simulink model "gm_comm8qamtxrxhdl"  (R2025b)
settings: Solver=FixedStepDiscrete  StartTime=0.0  StopTime=20000*qam_params.symbolPeriod  RelTol=1e-3
PreLoadFcn:
  | qam_params = comm8qamtxrxhdl_init;
InitFcn:
  | qam_params = comm8qamtxrxhdl_init;
libraries: simulink x16, hdlmdlgenlib x7, hdlsllib x7, commchan3 x1, commrflib2 x1, dspsigops x1, dsphdlsigops2 x1, dspmlti4 x1, commdigbbndam3 x1, commsequence2 x1
(part 1 of 3)
settings Model: Creator=The MathWorks, Inc.  LastModifiedBy=Ubaid
settings SolverCC: AlgebraicLoopSolver=TrustRegion  MaxZcPerStep=1.0
settings DataIOCC: LimitDataPoints=on  SaveFormat=Array  SaveOutput=off  SaveTime=off  ReturnWorkspaceOutputs=off
settings OptimizationCC: BlockReduction=off  ConditionallyExecuteInputs=off  DefaultParameterBehavior=Inlined  ReuseModelBlockBuffer=off  LifeSpan=inf
settings DebuggingCC: AlgebraicLoopMsg=error  ArtificialAlgebraicLoopMsg=none  UnderspecifiedInitializationDetection=Classic  MergeDetectMultiDrivingBlocksExec=none  SolverPrmCheckMsg=warning  InheritedTsInSrcMsg=none  MultiTaskDSMMsg=warning  MultiTaskCondExecSysMsg=none  SingleTaskRateTransMsg=error  IntegerOverflowMsg=none  ParameterPrecisionLossMsg=none  UnconnectedInputMsg=warning  UnconnectedOutputMsg=warning  UnconnectedLineMsg=warning  AllowSymbolicDim=off  StateNameClashWarn=warning  SFUnexpectedBacktrackingDiag=warning  SFNoUnconditionalDefaultTransitionDiag=warning  SFExecutionAtInitializationDiag=none  IntegerSaturationMsg=none  ArithmeticOperatorsInVariantConditions=warning
settings HardwareCC: ProdBitPerPointer=32.0  ProdBitPerSizeT=32.0  ProdBitPerPtrDiffT=32.0  ProdLargestAtomicFloat=None  ProdIntDivRoundTo=Undefined  ProdEndianess=Unspecified  ProdWordSize=32.0  ProdHWDeviceType=ASIC/FPGA->ASIC/FPGA  ProdEqTarget=off
settings ModelReferenceCC: EnableRefExpFcnMdlSchedulingChecks=on  PropagateSignalLabelsOutOfModel=off
settings SFSimCC: SimUseLocalCustomCode=off  CustomCodeUndefinedFunction=UseInterfaceOnly
settings RTWCC: RTWUseLocalCustomCode=off  GPUComputeCapability=3.5  DLArmComputeVersion=19.05
settings CodeAppCC: StateflowObjectComments=on
settings GRTTargetCC: TargetLangStandard=C89/C90 (ANSI)
settings ConfigComp: CovMetricSettings=dw  CovSaveCumulativeToWorkspaceVar=on  CovSaveSingleToWorkspaceVar=on  CovExternalEMLEnable=off  CovSFcnEnable=off

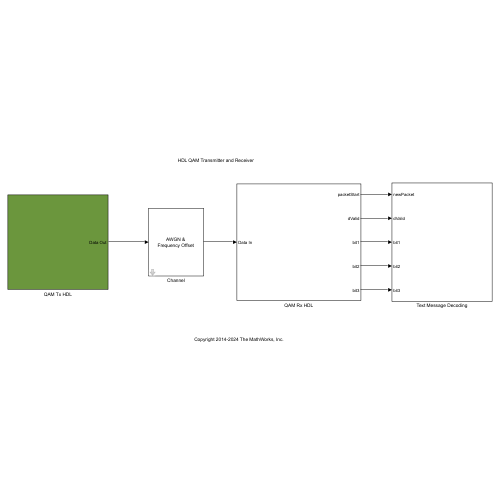
[thumbnail: Simulink's stored preview of the top-level diagram]
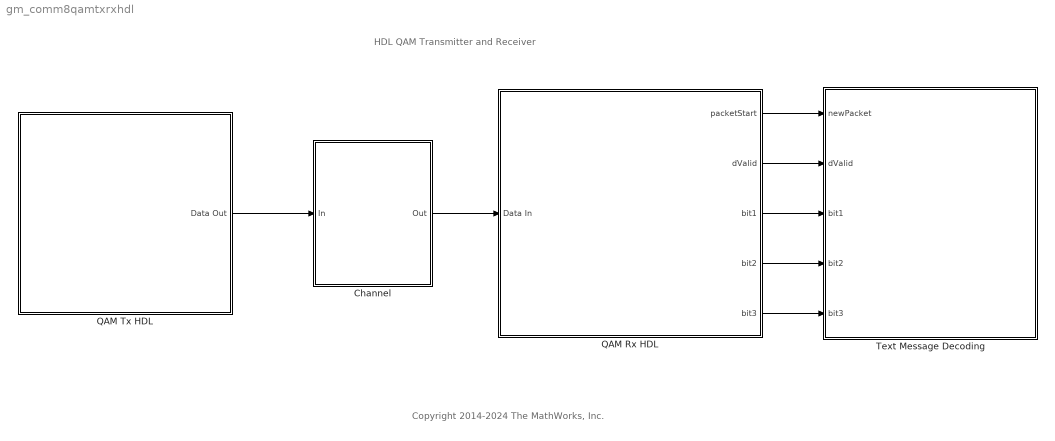
== system gm_comm8qamtxrxhdl ==
  note: HDL QAM Transmitter and Receiver
  note: Copyright 2014-2024 The MathWorks, Inc.
  Channel : Subsystem  mask{Poff=qam_params.phaseOffset, Foff=qam_params.frequencyOffset, EbNo=qam_params.EbNo, Chan_Gain=qam_params.channelGain, Chan_Delay=qam_params.channelDelay}
      mask prompts: Poff "Phase offset (deg)"; Foff "Frequency offset (Hz)"; EbNo "Eb/No"; Chan_Gain "Channel Gain"; Chan_Delay "Channel Delay"
      mask Display: disp('AWGN &\nFrequency Offset');
  QAM Rx HDL : Subsystem
  QAM Tx HDL : Subsystem
  Text Message Decoding : Subsystem
  wires:
  QAM Tx HDL/1(Data Out) -> Channel/1(In)
  Channel/1(Out) -> QAM Rx HDL/1(Data In)
  QAM Rx HDL/2(dValid) -> Text Message Decoding/2(dValid)
  QAM Rx HDL/5(bit3) -> Text Message Decoding/5(bit3)
  QAM Rx HDL/4(bit2) -> Text Message Decoding/4(bit2)
  QAM Rx HDL/3(bit1) -> Text Message Decoding/3(bit1)
  QAM Rx HDL/1(packetStart) -> Text Message Decoding/1(newPacket)

== system gm_comm8qamtxrxhdl/Channel ==
  In : Inport
  AWGN Channel2 : commchan3/AWGN Channel  LegacyMode=on  NoiseMethod="Signal to noise ratio  (Eb/No)"  noiseMode="Signal to noise ratio  (SNR)"  EbNo=EbNo  EsNo=15  SNR=15  BitsPerSymbol=3  SignalPower=0.11  SpecifySymbolPeriod=off  SamplesPerSymbol=1  SymbolPeriod=1/qam_params.sampleRate  VarianceSource=Parameter  Variance=1  RandomStream=Global stream  Seed=67  SimulateUsing=Code generation
  Constant : Constant  Value=Chan_Delay  SampleTime=1/qam_params.sampleRate
  Data Type Conversion1 : DataTypeConversion  OutDataTypeStr=fixdt(1,16,15)  SaturateOnIntegerOverflow=off  RndMeth=Floor
  Data Type Conversion4 : DataTypeConversion  OutDataTypeStr=double  SaturateOnIntegerOverflow=off  RndMeth=Floor
  Gain : Gain  Gain=Chan_Gain
  Phase/ Frequency Offset1 : commrflib2/Phase// Frequency Offset  phaseOffset=Poff  freqPort=off  freqOffset=Foff
  Variable Fractional Delay : dspsigops/Variable Fractional Delay  mode=OBSOLETE  modeActive=Linear  L=4  FarrowL=4  R=10  alpha=1  dmax=56*4  ic=0  noDFT=off  fallbackFIR=Clip to the minimum value necessary for centered kernel  fallbackFarrow=Clip to the minimum value necessary for centered kernel  roundingMode=Zero  overflowMode=off
  Out : Outport  VectorParamsAs1DForOutWhenUnconnected=off
  wires:
  Gain/1 -> Data Type Conversion1/1
  Constant/1 -> Variable Fractional Delay/2
  Variable Fractional Delay/1 -> AWGN Channel2/1
  Phase/ Frequency Offset1/1 -> Variable Fractional Delay/1
  Data Type Conversion4/1 -> Phase/ Frequency Offset1/1
  Data Type Conversion1/1 -> Out/1
  AWGN Channel2/1 -> Gain/1
  In/1 -> Data Type Conversion4/1

== system gm_comm8qamtxrxhdl/QAM Rx HDL ==
  Data In : Inport  OutDataTypeStr=fixdt(1, 16, 15)  PortDimensions=1  SampleTime=2.5e-07
      settings: SignalType=complex
  AND : Logic  AllPortsSameDT=off  OutDataTypeStr=boolean  SampleTime=5e-07
  Automatic Gain Control : Subsystem  mask{AGC_Ref=double(0.23), AGC_Gain=double(0.001)}
      mask prompts: AGC_Ref "Target Amplitude"; AGC_Gain "AGC Loop Gain"
  Coarse Frequency Offset Correction : Subsystem
  Delay3 : Delay  DelayLength=double(2)  InitialCondition=0  SampleTime=5e-07
  Demodulate : Subsystem
  Magnitude & Phase Recovery : Subsystem  mask{PreAmb=reshape(complex(double([0.75+0.25i;0.75+0.25i;0.75+0.25i;0.75+0.25i;0.75+0.25i;-0.75-0.25i;-0.75-0.25i;0.75+0.25i;0.75+0.25i;-0.75-0.25i;0.75+0.25i;-0.75-0.25i;0.75+0.25i;0.75+0.25i])), [1  14]), threshold=double(1.1), LMS_Step=double(0.25)}
      mask prompts: PreAmb "Preamble symbols"; LMS_Step "LMS step size"
  Timing Recovery : Subsystem
  packetStart : Outport  SampleTime=5e-07  VectorParamsAs1DForOutWhenUnconnected=off
  dValid : Outport  Port=2  SampleTime=5e-07  VectorParamsAs1DForOutWhenUnconnected=off
  bit1 : Outport  Port=3  SampleTime=5e-07  VectorParamsAs1DForOutWhenUnconnected=off
  bit2 : Outport  Port=4  SampleTime=5e-07  VectorParamsAs1DForOutWhenUnconnected=off
  bit3 : Outport  Port=5  SampleTime=5e-07  VectorParamsAs1DForOutWhenUnconnected=off
  wires:
  Data In/1 -> Automatic Gain Control/1(x)
  Magnitude & Phase Recovery/1(valid) -> AND/2
  Timing Recovery/2(dataOut) -> Magnitude & Phase Recovery/1(Input)
  Automatic Gain Control/1(y) -> Coarse Frequency Offset Correction/1(dataIn)
  Demodulate/1(Valid) -> dValid/1
  Coarse Frequency Offset Correction/1(dataOut) -> Timing Recovery/1(dataIn)
  Magnitude & Phase Recovery/2(corrected) -> Demodulate/2(Symbols In)
  AND/1 -> Demodulate/1(valid_in)
  Timing Recovery/1(validOut) -> AND/1, Magnitude & Phase Recovery/2(Enable)
  Demodulate/3(Bit2) -> bit2/1
  Magnitude & Phase Recovery/3(isPreamble) -> Delay3/1
  Delay3/1 -> packetStart/1
  Demodulate/2(Bit1) -> bit1/1
  Demodulate/4(Bit3) -> bit3/1

== system gm_comm8qamtxrxhdl/QAM Tx HDL ==
  " Zero" : Constant  Value=complex(0,0)  OutDataTypeStr=fixdt(1,16,15)  SampleTime=qam_params.symbolPeriod
  Data Generation & Packetization : Subsystem
  Input Mux : MultiPortSwitch  DataPortOrder=Zero-based contiguous  Inputs=2  zeroidx=on  SaturateOnIntegerOverflow=off  InputSameDT=off
  Pipeline{1..5} (5 alike) : Delay  DelayLength=1  InitialCondition=0
  Pulse Shaping : Subsystem
  Symbol Mapping : Subsystem
  Data Out : Outport  VectorParamsAs1DForOutWhenUnconnected=off
  wires:
  Pulse Shaping/1(dataOut) -> Pipeline5/1
  Input Mux/1 -> Pulse Shaping/1(dataIn)
  Symbol Mapping/1(Valid out) -> Pipeline3/1
  Symbol Mapping/2(Symbol Out) -> Pipeline4/1
  Pipeline2/1 -> Symbol Mapping/2(Integer In)
  Data Generation & Packetization/2(Raw Data) -> Pipeline2/1
  Data Generation & Packetization/1(Valid Out) -> Pipeline1/1
  " Zero"/1 -> Input Mux/2
  Pipeline3/1 -> Input Mux/1
  Pipeline1/1 -> Symbol Mapping/1(Valid In)
  Pipeline5/1 -> Data Out/1
  Pipeline4/1 -> Input Mux/3

== system gm_comm8qamtxrxhdl/Text Message Decoding ==
  newPacket : Inport
  dValid : Inport  Port=2
  bit1 : Inport  Port=3
  bit2 : Inport  Port=4
  bit3 : Inport  Port=5
  " " : MATLAB Function  TreatAsAtomicUnit=on
  Descramble and Print : Subsystem  TreatAsAtomicUnit=on
  wires:
  newPacket/1 -> " "/1(newPacket)
  dValid/1 -> " "/2(dValid)
  bit3/1 -> " "/5(bit3)
  " "/1(RxGo) -> Descramble and Print/Enable
  " "/2(framed_data) -> Descramble and Print/1(In1)
  bit2/1 -> " "/4(bit2)
  bit1/1 -> " "/3(bit1)

== system gm_comm8qamtxrxhdl/QAM Rx HDL/Automatic Gain Control ==
  x : Inport  OutDataTypeStr=fixdt(1, 16, 15)  PortDimensions=1  SampleTime=2.5e-07
      settings: SignalType=complex
  Delay : Delay  DelayLength=double(2)  InitialCondition=0  SampleTime=2.5e-07
  Delay1 : Delay  DelayLength=double(2)  InitialCondition=0  SampleTime=2.5e-07
  Delay2 : Delay  DelayLength=double(1)  InitialCondition=0  SampleTime=2.5e-07
  Delay4 : Delay  DelayLength=double(2)  InitialCondition=0  SampleTime=2.5e-07
  Loop gain : Constant  Value=0.001007080078125  OutDataTypeStr=fixdt(1, 16, 15)  SampleTime=2.5e-07
  Product : Product  Inputs=**  OutDataTypeStr=fixdt(1, 16, 15)  SaturateOnIntegerOverflow=on  SampleTime=2.5e-07
  Product1 : Product  Inputs=**  OutDataTypeStr=fixdt(1, 16, 15)  SaturateOnIntegerOverflow=on  SampleTime=2.5e-07
  Reference : Constant  Value=0.230010986328125  OutDataTypeStr=fixdt(1, 16, 15)  SampleTime=2.5e-07
  Sum : Sum  OutDataTypeStr=fixdt(1, 24, 15)  AccumDataTypeStr=fixdt(1, 24, 15)  SaturateOnIntegerOverflow=on  SampleTime=2.5e-07
  Sum1 : Sum  Inputs=+-  OutDataTypeStr=fixdt(1, 16, 14)  AccumDataTypeStr=fixdt(1, 18, 15)  SampleTime=2.5e-07
  Unit Delay : Delay  DelayLength=double(1)  InitialCondition=0.5  SampleTime=2.5e-07
  power : Subsystem
  y : Outport  PortDimensions=1  SampleTime=2.5e-07  VectorParamsAs1DForOutWhenUnconnected=off
  wires:
  Delay2/1 -> Product1/1
  Reference/1 -> Sum1/1
  power/1(Out1) -> Sum1/2
  x/1 -> Delay1/1
  Sum1/1 -> Delay2/1
  Product1/1 -> Delay4/1
  Loop gain/1 -> Product1/2
  Delay4/1 -> Sum/2
  Unit Delay/1 -> Product/2, Sum/1
  Delay1/1 -> Product/1
  Sum/1 -> Unit Delay/1
  Product/1 -> Delay/1
  Delay/1 -> power/1(In1), y/1

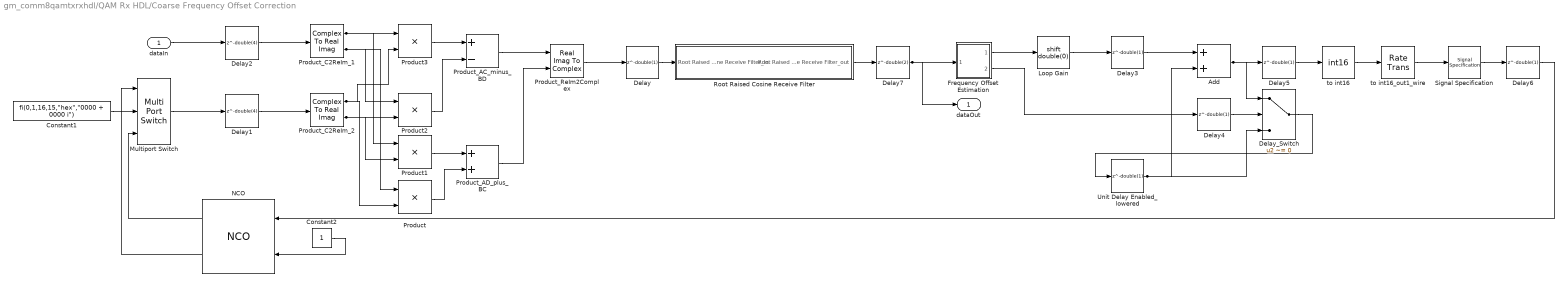
== system gm_comm8qamtxrxhdl/QAM Rx HDL/Coarse Frequency Offset Correction ==
  dataIn : Inport  OutDataTypeStr=fixdt(1, 16, 15)  PortDimensions=1  SampleTime=2.5e-07
      settings: SignalType=complex
  Add : Sum  OutDataTypeStr=fixdt(1, 16, 3)  AccumDataTypeStr=fixdt(1, 16, 3)  SampleTime=5e-07
  Constant1 : Constant  Value="fi(0,1,16,15,\"hex\",\"0000 + 0000 i\")"  OutDataTypeStr=fixdt(1, 16, 15)  SampleTime=2.5e-07
  Constant2 : Constant  OutDataTypeStr=boolean  SampleTime=2.5e-07
  Delay : Delay  DelayLength=double(1)  InitialCondition=0  SampleTime=2.5e-07
  Delay1 : Delay  DelayLength=double(4)  InitialCondition=0  SampleTime=2.5e-07
  Delay2 : Delay  DelayLength=double(4)  InitialCondition=0  SampleTime=2.5e-07
  Delay3 : Delay  DelayLength=double(1)  InitialCondition=0  SampleTime=5e-07
  Delay4 : Delay  DelayLength=double(1)  InitialCondition=0  SampleTime=5e-07
  Delay5 : Delay  DelayLength=double(1)  InitialCondition=0  SampleTime=5e-07
  Delay6 : Delay  DelayLength=double(1)  InitialCondition=0  SampleTime=2.5e-07
  Delay7 : Delay  DelayLength=double(2)  InitialCondition=0  SampleTime=5e-07
  Delay_Switch : Switch  Criteria=u2 ~= 0  Threshold=double(0)  OutDataTypeStr=fixdt(1, 16, 3)  SampleTime=5e-07  SaturateOnIntegerOverflow=off  InputSameDT=off
  Frequency Offset Estimation : Subsystem  mask{M=double(64), N=double(256), avFilterCoeffs=double(0)}
      mask prompts: M "M (Luise Parameter)"; N "N (Luise Parameter)"; avFilterCoeffs "Filter Coeffs"
      mask init:
      | M = double(64);
      | N = double(256);
      | avFilterCoeffs = reshape(double([0.00390625;0.00390625;0.00390625;0.00390625;0.00390625;0.00390625;0.00390625;0.00390625;0.00390625;0.00390625;0.00390625;0.00390625;0.00390625;0.00390625;0.00390625;0.00390625;0.00390625;0.00390625;0.00390625;0.00390625;0.00390625;0.00390625;0.00390625;0.00390625;0.00390625;0.00390625;0.00390625;0.00390625;0.00390625;0.00390625;0.00390625;0.00390625;0.00390625;0.00390625;0.00390625;0.00390625;0.00390625;0.00390625;0.00390625;0.00390625;0.00390625;0.00390625;0.00390625;0.00390625;0.00390625;0.00390625;0.00390625;0.00390625;0.00390625;0.00390625;0.00390625;0.00390625;0.00390625;0.00390625;0.00390625;0.00390625;0.00390625;0.00390625;0.00390625;0.00390625;0.00390625;0.00390625;0.00390625;0.00390625]), [1  64]);
  Loop Gain : ArithShift  BitShiftNumber=double(0)  BinPtShiftNumber=double(-3)
  Multiport Switch : MultiPortSwitch  DataPortOrder=Zero-based contiguous  Inputs=2  DiagnosticForDefault=None  zeroidx=on  OutDataTypeStr=fixdt(1, 16, 15)  SampleTime=2.5e-07  SaturateOnIntegerOverflow=off  InputSameDT=off
  NCO : dsphdlsigops2/NCO  PhaseIncrementSource=Input port  PhaseIncrement=100  PhaseOffsetSource=Property  PhaseOffset=0  DitherSource=Property  NumDitherBits=4  SamplesPerFrame=1  LUTCompress=off  ResetAction=off  Waveform=Complex exponential  PhasePort=off  SimulateUsing=Code generation  AccumulatorWL=16  PhaseQuantization=on  NumQuantizerAccumulatorBits=16  OutputDataType=Binary point scaling  OutputWL=16  OutputFL=15
  Product{,1..3} (4 alike) : Product  Inputs=**  OutDataTypeStr=fixdt(1, 16, 15)  SampleTime=2.5e-07
  Product_AC_minus_BD : Sum  Inputs=+-  OutDataTypeStr=fixdt(1, 16, 15)  SampleTime=2.5e-07
  Product_AD_plus_BC : Sum  OutDataTypeStr=fixdt(1, 16, 15)  SampleTime=2.5e-07
  Product_C2ReIm_1 : ComplexToRealImag  SampleTime=2.5e-07
  Product_C2ReIm_2 : ComplexToRealImag  SampleTime=2.5e-07
  Product_ReIm2Complex : RealImagToComplex  SampleTime=2.5e-07
  Root Raised Cosine Receive Filter : Subsystem
  Signal Specification : SignalSpecification  OutDataTypeStr=int16  Dimensions=1
  Unit Delay Enabled_lowered : Delay  DelayLength=double(1)  InitialCondition=0  SampleTime=5e-07
  to int16 : DataTypeConversion  OutDataTypeStr=int16  SampleTime=5e-07  SaturateOnIntegerOverflow=off  RndMeth=Floor
  to int16_out1_wire : RateTransition  Integrity=off  Deterministic=off  OutPortSampleTimeOpt=Multiple of input port sample time  OutPortSampleTimeMultiple=1/2
  dataOut : Outport  SampleTime=5e-07  VectorParamsAs1DForOutWhenUnconnected=off
  wires:
  Delay1/1 -> Product_C2ReIm_2/1
  Add/1 -> Delay_Switch/1, Delay5/1
  Constant1/1 -> Multiport Switch/2
  dataIn/1 -> Delay2/1
  Delay2/1 -> Product_C2ReIm_1/1
  Multiport Switch/1 -> Delay1/1
  Product/1 -> Product_AD_plus_BC/2
  NCO/2 -> Multiport Switch/1
  NCO/1 -> Multiport Switch/3
  Product_C2ReIm_1/1 -> Product3/1, Product1/1
  Product_C2ReIm_1/2 -> Product2/1, Product/1
  Product_C2ReIm_2/1 -> Product/2, Product3/2
  Product_C2ReIm_2/2 -> Product2/2, Product1/2
  Constant2/1 -> NCO/2
  Product3/1 -> Product_AC_minus_BD/1
  Product2/1 -> Product_AC_minus_BD/2
  Product1/1 -> Product_AD_plus_BC/1
  Product_AC_minus_BD/1 -> Product_ReIm2Complex/1
  Signal Specification/1 -> Delay6/1
  Product_AD_plus_BC/1 -> Product_ReIm2Complex/2
  Product_ReIm2Complex/1 -> Delay/1
  Delay/1 -> Root Raised Cosine Receive Filter/1(Root Raised Cosine Receive Filter_In)
  Root Raised Cosine Receive Filter/1(Root Raised Cosine Receive Filter_out) -> Delay7/1
  Delay7/1 -> dataOut/1, Frequency Offset Estimation/1(dataIn)
  Frequency Offset Estimation/1(Estimate) -> Loop Gain/1
  to int16/1 -> to int16_out1_wire/1
  Delay5/1 -> to int16/1
  Frequency Offset Estimation/2(Estimate Valid) -> Delay4/1
  Loop Gain/1 -> Delay3/1
  Delay3/1 -> Add/1
  Unit Delay Enabled_lowered/1 -> Delay_Switch/3, Add/2
  Delay4/1 -> Delay_Switch/2
  Delay_Switch/1 -> Unit Delay Enabled_lowered/1
  to int16_out1_wire/1 -> Signal Specification/1
  Delay6/1 -> NCO/1

== system gm_comm8qamtxrxhdl/QAM Rx HDL/Demodulate ==
  valid_in : Inport  OutDataTypeStr=boolean  PortDimensions=1  SampleTime=5e-07
  Symbols In : Inport  Port=2  OutDataTypeStr=fixdt(1, 16, 14)  PortDimensions=1  SampleTime=5e-07
      settings: SignalType=complex
  Delay{1..4} (4 alike) : Delay  DelayLength=double(1)  InitialCondition=0  SampleTime=5e-07
  Rectangular QAM Demodulator Baseband : Subsystem
  Shift Arithmetic : ArithShift  BitShiftNumber=double(0)  BinPtShiftNumber=double(2)
  t : Demux  Outputs=3
  Valid : Outport  SampleTime=5e-07  VectorParamsAs1DForOutWhenUnconnected=off
  Bit1 : Outport  Port=2  SampleTime=5e-07  VectorParamsAs1DForOutWhenUnconnected=off
  Bit2 : Outport  Port=3  SampleTime=5e-07  VectorParamsAs1DForOutWhenUnconnected=off
  Bit3 : Outport  Port=4  SampleTime=5e-07  VectorParamsAs1DForOutWhenUnconnected=off
  wires:
  valid_in/1 -> Delay3/1
  Symbols In/1 -> Shift Arithmetic/1
  Delay3/1 -> Delay2/1
  Delay4/1 -> Rectangular QAM Demodulator Baseband/1(u)
  Rectangular QAM Demodulator Baseband/1(y) -> Delay1/1
  Shift Arithmetic/1 -> Delay4/1
  Delay1/1 -> t/1
  Delay2/1 -> Valid/1
  t/3 -> Bit3/1
  t/2 -> Bit2/1
  t/1 -> Bit1/1

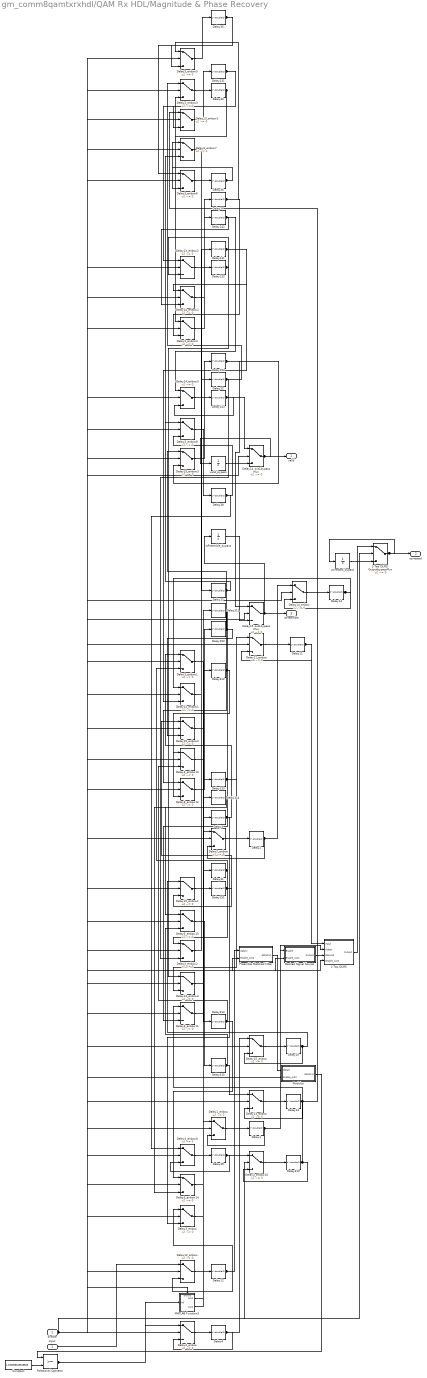
== system gm_comm8qamtxrxhdl/QAM Rx HDL/Magnitude & Phase Recovery ==
  Input : Inport  OutDataTypeStr=fixdt(1, 16, 15)  PortDimensions=1  SampleTime=5e-07
      settings: SignalType=complex
  Enable : Inport  Port=2  OutDataTypeStr=boolean  SampleTime=5e-07
  1-Tap DLMS : Subsystem
  1-Tap DLMS_OutputbypassMux : Switch  Criteria=u2 ~= 0  Threshold=double(0)  OutDataTypeStr=fixdt(1, 16, 14)  SampleTime=5e-07  SaturateOnIntegerOverflow=off  InputSameDT=off
  Constant : Constant  Value=1.100006103515625  OutDataTypeStr=fixdt(1, 18, 15)  SampleTime=5e-07
  Delay{1..4,11..15,31..39,131..133,141..143,151..153,310..315} (33 alike) : Delay  DelayLength=double(1)  InitialCondition=0
  Delay11_enbsw : Switch  Criteria=u2 ~= 0  Threshold=double(0)  OutDataTypeStr=fixdt(1, 16, 15)  SampleTime=5e-07  SaturateOnIntegerOverflow=off  InputSameDT=off
  Delay12_enbsw : Switch  Criteria=u2 ~= 0  Threshold=double(0)  OutDataTypeStr=fixdt(1, 16, 15)  SampleTime=5e-07  SaturateOnIntegerOverflow=off  InputSameDT=off
  Delay13_enbsw{,1..3} (4 alike) : Switch  Criteria=u2 ~= 0  Threshold=double(0)  OutDataTypeStr=fixdt(1, 16, 15)  SampleTime=5e-07  SaturateOnIntegerOverflow=off  InputSameDT=off
  Delay14_enbsw{,1..3} (4 alike) : Switch  Criteria=u2 ~= 0  Threshold=double(0)  OutDataTypeStr=boolean  SampleTime=5e-07  SaturateOnIntegerOverflow=off  InputSameDT=off
  Delay14_out1bypassMux : Switch  Criteria=u2 ~= 0  Threshold=double(0)  OutDataTypeStr=boolean  SampleTime=5e-07  SaturateOnIntegerOverflow=off  InputSameDT=off
  Delay15_enbsw{,1..3} (4 alike) : Switch  Criteria=u2 ~= 0  Threshold=double(0)  OutDataTypeStr=boolean  SampleTime=5e-07  SaturateOnIntegerOverflow=off  InputSameDT=off
  Delay15_out1bypassMux : Switch  Criteria=u2 ~= 0  Threshold=double(0)  OutDataTypeStr=boolean  SampleTime=5e-07  SaturateOnIntegerOverflow=off  InputSameDT=off
  Delay1_enbsw : Switch  Criteria=u2 ~= 0  Threshold=double(0)  OutDataTypeStr=boolean  SampleTime=5e-07  SaturateOnIntegerOverflow=off  InputSameDT=off
  Delay2_enbsw : Switch  Criteria=u2 ~= 0  Threshold=double(0)  OutDataTypeStr=boolean  SampleTime=5e-07  SaturateOnIntegerOverflow=off  InputSameDT=off
  Delay3_enbsw{,1..15} (16 alike) : Switch  Criteria=u2 ~= 0  Threshold=double(0)  OutDataTypeStr=fixdt(1, 16, 15)  SampleTime=5e-07  SaturateOnIntegerOverflow=off  InputSameDT=off
  Delay4_enbsw : Switch  Criteria=u2 ~= 0  Threshold=double(0)  OutDataTypeStr=boolean  SampleTime=5e-07  SaturateOnIntegerOverflow=off  InputSameDT=off
  Desired Signal Source : Subsystem
  MATLAB Function3 : Subsystem
      settings: MinAlgLoopOccurrences=on
  Modulus : Subsystem
  Preamble Matched Filter : Subsystem
  Relational Operator : RelationalOperator  OutDataTypeStr=boolean  SampleTime=5e-07
  corrected_bypass : UnitDelay  InitialCondition="fi(0,1,16,14,\"hex\",\"0000\")"  SampleTime=5e-07
  isPreamble_bypass : UnitDelay  SampleTime=5e-07
  valid_bypass : UnitDelay  SampleTime=5e-07
  valid : Outport  SampleTime=5e-07  InitialOutput=0  VectorParamsAs1DForOutWhenUnconnected=off
  corrected : Outport  Port=2  SampleTime=5e-07  InitialOutput=0  VectorParamsAs1DForOutWhenUnconnected=off
  isPreamble : Outport  Port=3  SampleTime=5e-07  InitialOutput=0  VectorParamsAs1DForOutWhenUnconnected=off
  wires:
  Delay3_enbsw12/1 -> Delay312/1
  Delay15_enbsw2/1 -> Delay152/1
  Delay13_enbsw2/1 -> Delay132/1
  Delay3_enbsw4/1 -> Delay34/1
  Delay3_enbsw5/1 -> Delay35/1
  Delay4_enbsw/1 -> Delay4/1
  Delay3_enbsw9/1 -> Delay39/1
  Delay15_enbsw3/1 -> Delay153/1
  Delay38/1 -> Delay3_enbsw9/1, Delay3_enbsw8/3
  corrected_bypass/1 -> 1-Tap DLMS_OutputbypassMux/3
  Delay14_out1bypassMux/1 -> valid_bypass/1, valid/1
  Delay3_enbsw13/1 -> Delay313/1
  Delay3_enbsw11/1 -> Delay311/1
  Delay15_enbsw1/1 -> Delay151/1
  Delay3_enbsw6/1 -> Delay36/1
  Constant/1 -> Relational Operator/2
  Delay15_enbsw/1 -> Delay15/1
  Delay3_enbsw7/1 -> Delay37/1
  Delay1_enbsw/1 -> Delay1/1
  Delay12/1 -> Delay12_enbsw/3, Delay3_enbsw/1, Preamble Matched Filter/1(dataIn)
  1-Tap DLMS/1(Output) -> 1-Tap DLMS_OutputbypassMux/1
  Delay1/1 -> Delay1_enbsw/3, 1-Tap DLMS/2(Adapt), Desired Signal Source/1(Enable)
  Delay3_enbsw1/1 -> Delay31/1
  Delay13_enbsw3/1 -> Delay133/1
  MATLAB Function3/2(out1) -> Delay1_enbsw/1
  Delay3_enbsw2/1 -> Delay32/1
  Delay11_enbsw/1 -> Delay11/1
  Delay13_enbsw1/1 -> Delay131/1
  Delay3_enbsw3/1 -> Delay33/1
  Delay143/1 -> Delay14_out1bypassMux/1, Delay14_enbsw3/3
  1-Tap DLMS_OutputbypassMux/1 -> corrected/1, corrected_bypass/1
  Delay3_enbsw8/1 -> Delay38/1
  Delay39/1 -> Delay3_enbsw9/3, Delay3_enbsw10/1
  MATLAB Function3/1(out0) -> Delay2_enbsw/1
  Delay153/1 -> Delay15_out1bypassMux/1, Delay15_enbsw3/3
  Delay14_enbsw3/1 -> Delay143/1
  Delay13_enbsw/1 -> Delay13/1
  Delay14_enbsw2/1 -> Delay142/1
  Delay3_enbsw15/1 -> Delay315/1
  valid_bypass/1 -> Delay14_out1bypassMux/3
  Delay313/1 -> Delay3_enbsw13/3, Delay3_enbsw14/1
  Delay3_enbsw/1 -> Delay3/1
  Delay3_enbsw14/1 -> Delay314/1
  Preamble Matched Filter/1(dataOut) -> Modulus/1(dataIn)
  Relational Operator/1 -> MATLAB Function3/1(in0), Delay4_enbsw/1
  Delay14_enbsw1/1 -> Delay141/1
  Delay15_out1bypassMux/1 -> isPreamble_bypass/1, isPreamble/1
  Delay3_enbsw10/1 -> Delay310/1
  Enable/1 -> MATLAB Function3/Enable, Modulus/2(Enable_out2), 1-Tap DLMS/4(Enable_out2), 1-Tap DLMS_OutputbypassMux/2, Delay14_out1bypassMux/2, Delay3_enbsw10/2, Delay2_enbsw/2, Desired Signal Source/2(Enable_out2), Delay1_enbsw/2, Delay13_enbsw/2, Delay14_enbsw/2, Delay15_out1bypassMux/2, Preamble Matched Filter/2(Enable_out2), Delay3_enbsw11/2, Delay4_enbsw/2, Delay3_enbsw14/2, Delay12_enbsw/2, Delay14_enbsw3/2, Delay3_enbsw6/2, Delay15_enbsw3/2, Delay3_enbsw/2, Delay3_enbsw1/2, Delay3_enbsw2/2, Delay3_enbsw3/2, Delay3_enbsw5/2, Delay3_enbsw7/2, Delay3_enbsw8/2, Delay3_enbsw12/2, Delay3_enbsw15/2, Delay3_enbsw13/2, Delay13_enbsw1/2, Delay13_enbsw2/2, Delay13_enbsw3/2, Delay14_enbsw1/2, Delay15_enbsw1/2, Delay15_enbsw2/2, Delay14_enbsw2/2, Delay3_enbsw9/2, Delay3_enbsw4/2, Delay11_enbsw/2, Delay15_enbsw/2
  Delay14_enbsw/1 -> Delay14/1
  Delay36/1 -> Delay3_enbsw7/1, Delay3_enbsw6/3
  Delay310/1 -> Delay3_enbsw11/1, Delay3_enbsw10/3
  isPreamble_bypass/1 -> Delay15_out1bypassMux/3
  Delay12_enbsw/1 -> Delay12/1
  Delay2_enbsw/1 -> Delay2/1
  Desired Signal Source/1(Output) -> 1-Tap DLMS/3(Desired)
  Input/1 -> Delay12_enbsw/1
  Delay35/1 -> Delay3_enbsw5/3, Delay3_enbsw6/1
  Delay4/1 -> Delay4_enbsw/3, Delay15_enbsw/1
  Delay11/1 -> Delay11_enbsw/3, 1-Tap DLMS/1(Input)
  Delay315/1 -> Delay3_enbsw15/3, Delay13_enbsw/1
  Delay2/1 -> Delay2_enbsw/3, Delay14_enbsw/1
  Delay133/1 -> Delay13_enbsw3/3, Delay11_enbsw/1
  Delay131/1 -> Delay13_enbsw2/1, Delay13_enbsw1/3
  Delay151/1 -> Delay15_enbsw1/3, Delay15_enbsw2/1
  Delay13/1 -> Delay13_enbsw/3, Delay13_enbsw1/1
  Delay15/1 -> Delay15_enbsw1/1, Delay15_enbsw/3
  Delay32/1 -> Delay3_enbsw3/1, Delay3_enbsw2/3
  Delay141/1 -> Delay14_enbsw2/1, Delay14_enbsw1/3
  Delay37/1 -> Delay3_enbsw8/1, Delay3_enbsw7/3
  Delay31/1 -> Delay3_enbsw2/1, Delay3_enbsw1/3
  Delay142/1 -> Delay14_enbsw2/3, Delay14_enbsw3/1
  Delay34/1 -> Delay3_enbsw4/3, Delay3_enbsw5/1
  Delay3/1 -> Delay3_enbsw1/1, Delay3_enbsw/3
  Delay312/1 -> Delay3_enbsw12/3, Delay3_enbsw13/1
  Delay132/1 -> Delay13_enbsw3/1, Delay13_enbsw2/3
  Delay14/1 -> Delay14_enbsw1/1, Delay14_enbsw/3
  Delay152/1 -> Delay15_enbsw2/3, Delay15_enbsw3/1
  Delay33/1 -> Delay3_enbsw4/1, Delay3_enbsw3/3
  Delay311/1 -> Delay3_enbsw12/1, Delay3_enbsw11/3
  Delay314/1 -> Delay3_enbsw14/3, Delay3_enbsw15/1
  Modulus/1(dataOut) -> Relational Operator/1

== system gm_comm8qamtxrxhdl/QAM Rx HDL/Timing Recovery ==
  dataIn : Inport  OutDataTypeStr=fixdt(1, 16, 15)  PortDimensions=1  SampleTime=5e-07
      settings: SignalType=complex
  Delay1 : Delay  DelayLength=double(1)  InitialCondition=0  SampleTime=5e-07
  Delay2 : Delay  DelayLength=double(1)  InitialCondition=0  SampleTime=5e-07
  Delay5 : Delay  DelayLength=double(6)  InitialCondition=0  SampleTime=5e-07
  Gain : Gain  Gain="fi(0,1,16,23,\"hex\",\"8000\")"  ParamDataTypeStr=fixdt(1, 16, 23)  OutDataTypeStr=fixdt(1, 16, 15)  SampleTime=5e-07
  Integer Delay3 : Delay  DelayLength=double(1)  InitialCondition=0  SampleTime=5e-07
  Integer Delay4 : Delay  DelayLength=double(1)  InitialCondition=0  SampleTime=5e-07
  Interpolation Control : Subsystem
  "Interpolation Filter " : Subsystem
  Timing Error Detector : Subsystem
  validOut : Outport  SampleTime=5e-07  VectorParamsAs1DForOutWhenUnconnected=off
  dataOut : Outport  Port=2  SampleTime=5e-07  VectorParamsAs1DForOutWhenUnconnected=off
  wires:
  Delay1/1 -> Interpolation Control/1(Delta)
  Timing Error Detector/1(e) -> Delay2/1
  Delay2/1 -> Gain/1
  Integer Delay3/1 -> "Interpolation Filter "/3(validIn)
  dataIn/1 -> Delay5/1
  Gain/1 -> Delay1/1
  Interpolation Control/1(Underflow) -> Integer Delay3/1
  Interpolation Control/2(mu) -> Integer Delay4/1
  Delay5/1 -> "Interpolation Filter "/1(dataIn)
  Integer Delay4/1 -> "Interpolation Filter "/2(mu)
  "Interpolation Filter "/1(dataOut) -> Timing Error Detector/1(In), dataOut/1
  "Interpolation Filter "/2(validOut) -> Timing Error Detector/2(strobe), validOut/1

== system gm_comm8qamtxrxhdl/QAM Tx HDL/Data Generation & Packetization ==
  Controller FSM : MATLAB Function  TreatAsAtomicUnit=on  SystemSampleTime=1/qam_params.bitRate
  Data Source : Subsystem
  Downsample : DownSample  N=3  RateOptions=Allow multirate processing
  Group Bits : Subsystem
  Pipeline : Delay  InitialCondition=0
  Pipeline1 : Delay  DelayLength=1  InitialCondition=0
  Pipeline2 : Delay  DelayLength=1  InitialCondition=0
  Valid : Constant  OutDataTypeStr=boolean  SampleTime=1/qam_params.bitRate
  Valid Out : Outport  VectorParamsAs1DForOutWhenUnconnected=off
  Raw Data : Outport  Port=2  VectorParamsAs1DForOutWhenUnconnected=off
  wires:
  Controller FSM/1(reset_preamble) -> Data Source/1(reset preamble)
  Controller FSM/2(load_preamble) -> Data Source/2(load preamble)
  Controller FSM/3(load_data) -> Data Source/3(load data)
  Group Bits/1(Integer Out) -> Raw Data/1
  Pipeline2/1 -> Group Bits/1(Bits In)
  Downsample/1 -> Valid Out/1
  Pipeline/1 -> Pipeline1/1
  Pipeline1/1 -> Downsample/1
  Valid/1 -> Pipeline/1
  Data Source/1(packet_bits) -> Pipeline2/1

== system gm_comm8qamtxrxhdl/QAM Tx HDL/Pulse Shaping ==
  dataIn : Inport
  RRC Interpolation Filter : dspmlti4/FIR Interpolation  FilterSource=Dialog parameters  PrivateCoeffs=0  h=qam_params.TransmitterFilterCoefficients  L=4  FilterObject=Htxrc  framing=Allow multirate processing  outputBufInitCond=0  roundingMode=Nearest  overflowMode=on  firstCoeffMode=Binary point scaling  firstCoeffWordLength=16  firstCoeffFracLength=15  firstCoeffDataTypeStr=fixdt(1,16,15)  firstCoeffMin=[]  firstCoeffMax=[]  firstCoeffLastDataTypeStr=fixdt(1,16,15)  prodOutputMode=Binary point scaling  prodOutputWordLength=16  prodOutputFracLength=15  prodOutputDataTypeStr=fixdt(1,16,15)  prodOutputLastDataTypeStr=fixdt(1,16,15)  accumMode=Binary point scaling  accumWordLength=16  accumFracLength=15  accumDataTypeStr=fixdt(1,16,15)  accumLastDataTypeStr=fixdt(1,16,15)  outputMode=Binary point scaling  outputWordLength=16  outputFracLength=15  outputDataTypeStr=fixdt(1,16,15)  outputMin=[]  outputMax=[]  outputLastDataTypeStr=fixdt(1,16,15)
  dataOut : Outport  VectorParamsAs1DForOutWhenUnconnected=off
  wires:
  dataIn/1 -> RRC Interpolation Filter/1
  RRC Interpolation Filter/1 -> dataOut/1

== system gm_comm8qamtxrxhdl/QAM Tx HDL/Symbol Mapping ==
  Valid In : Inport
  Integer In : Inport  Port=2
  Rectangular QAM Modulator Baseband : commdigbbndam3/Rectangular QAM Modulator Baseband  M=8  InType=Integer  Enc=Gray  Mapping=[0:15]  PowType=Min. distance between symbols  MinDist=0.5  AvgPow=.66  PeakPow=1.1  Ph=0  outDtype=Fixed-point  outWordLen=16  outUDDataType=sfix(16)  outFracLenMode=Best precision  outFracLen=15  outDataTypeStr=fixdt(1,16)  outLastDataTypeStr=fixdt(1,16)
  Valid out : Outport  VectorParamsAs1DForOutWhenUnconnected=off
  Symbol Out : Outport  Port=2  VectorParamsAs1DForOutWhenUnconnected=off
  wires:
  Valid In/1 -> Valid out/1
  Integer In/1 -> Rectangular QAM Modulator Baseband/1
  Rectangular QAM Modulator Baseband/1 -> Symbol Out/1

== system gm_comm8qamtxrxhdl/Text Message Decoding/Descramble and Print ==
  In1 : Inport
  Enable : EnablePort
  BitsToDecimal1 : MATLAB Function  TreatAsAtomicUnit=on
  Descrambler : commsequence2/Descrambler  M=2  poly=[1 1 1 0 1]  iniStaSource=Dialog Parameter  ini_sta=[0 0 0 0]  resetViaPort=off
  Selector : Selector  IndexOptions=Index vector (dialog)  Indices=[43:1:168]  OutputSizes=1
  Selector1 : Selector  IndexOptions=Index vector (dialog)  Indices=[1:1:126]  OutputSizes=1
  wires:
  Descrambler/1 -> Selector1/1
  Selector/1 -> Descrambler/1
  In1/1 -> Selector/1
  Selector1/1 -> BitsToDecimal1/1(u)

== system gm_comm8qamtxrxhdl/QAM Rx HDL/Automatic Gain Control/power ==
  In1 : Inport  OutDataTypeStr=fixdt(1, 16, 15)  PortDimensions=1  SampleTime=2.5e-07
      settings: SignalType=complex
  Complex to Real-Imag : ComplexToRealImag
  Delay : Delay  InitialCondition=0
  Delay1 : Delay  InitialCondition=0
  Delay2 : Delay  InitialCondition=0
  Product3 : Product  OutDataTypeStr=fixdt(1,16,15)  SaturateOnIntegerOverflow=on
  Product4 : Product  OutDataTypeStr=fixdt(1,16,15)  SaturateOnIntegerOverflow=on
  Sum1 : Sum  OutDataTypeStr=fixdt(1,16,14)  AccumDataTypeStr=fixdt(1,16,15)  SaturateOnIntegerOverflow=on
  Out1 : Outport  SampleTime=2.5e-07  VectorParamsAs1DForOutWhenUnconnected=off
  wires:
  Complex to Real-Imag/2 -> Product4/2, Product4/1
  In1/1 -> Complex to Real-Imag/1
  Product3/1 -> Delay/1
  Complex to Real-Imag/1 -> Product3/2, Product3/1
  Product4/1 -> Delay1/1
  Delay/1 -> Sum1/1
  Delay1/1 -> Sum1/2
  Sum1/1 -> Delay2/1
  Delay2/1 -> Out1/1

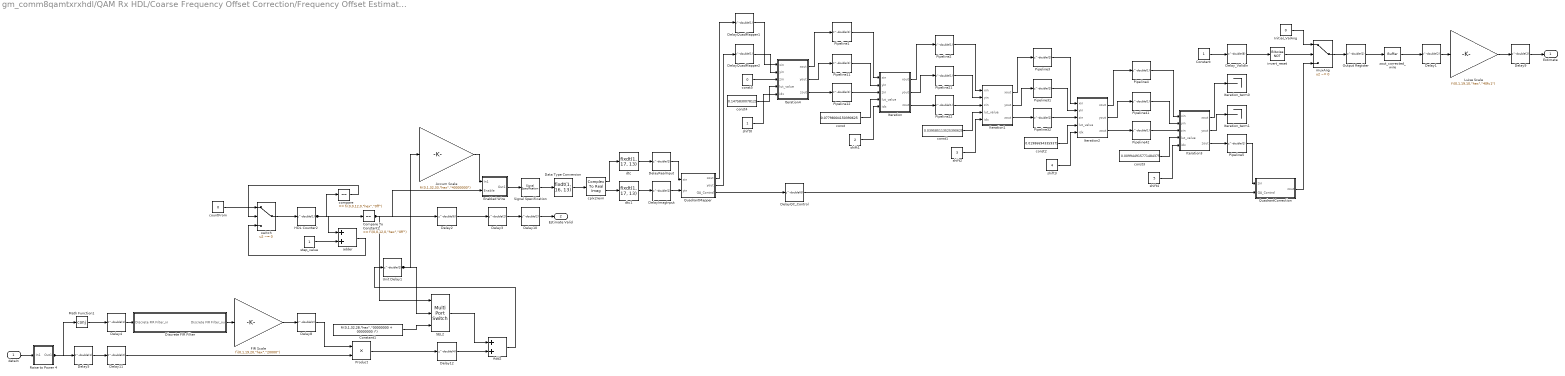
== system gm_comm8qamtxrxhdl/QAM Rx HDL/Coarse Frequency Offset Correction/Frequency Offset Estimation ==
  dataIn : Inport  OutDataTypeStr=fixdt(1, 16, 15)  PortDimensions=1  SampleTime=5e-07
      settings: SignalType=complex
  Accum Scale : Gain  Gain="fi(0,1,32,33,\"hex\",\"40000000\")"  ParamDataTypeStr=fixdt(1, 32, 33)  OutDataTypeStr=fixdt(1, 32, 31)  SampleTime=5e-07
  Add2 : Sum  OutDataTypeStr=fixdt(1, 32, 28)  AccumDataTypeStr=fixdt(1, 36, 31)  SampleTime=5e-07
  Compare To Constant2 : simulink/Logic and Bit Operations/Compare To Constant  relop===  const="fi(0,0,12,0,\"hex\",\"0ff\")"  OutDataTypeStr=boolean
  Constant : Constant  OutDataTypeStr=boolean  SampleTime=5e-07
  Constant1 : Constant  Value="fi(0,1,32,28,\"hex\",\"00000000 + 00000000 i\")"  OutDataTypeStr=fixdt(1, 32, 28)  SampleTime=5e-07
  Data Type Conversion : DataTypeConversion  OutDataTypeStr=fixdt(1, 16, 13)  SampleTime=5e-07  SaturateOnIntegerOverflow=off  RndMeth=Floor
  Delay{1,3,8..11} (6 alike) : Delay  DelayLength=double(2)  InitialCondition=0  SampleTime=5e-07
  Delay12 : Delay  DelayLength=double(4)  InitialCondition=0  SampleTime=5e-07
  Delay2 : Delay  DelayLength=double(6)  InitialCondition=0  SampleTime=5e-07
  Delay4 : Delay  DelayLength=double(1)  InitialCondition=0  SampleTime=5e-07
  Delay5 : Delay  DelayLength=double(1)  InitialCondition=0  SampleTime=5e-07
  DelayImagInput : Delay  DelayLength=double(1)  InitialCondition=0  SampleTime=5e-07
  DelayQC_Control : Delay  DelayLength=double(6)  InitialCondition=0  SampleTime=5e-07
  DelayQuadMapper1 : Delay  DelayLength=double(1)  InitialCondition=0  SampleTime=5e-07
  DelayQuadMapper2 : Delay  DelayLength=double(1)  InitialCondition=0  SampleTime=5e-07
  DelayRealInput : Delay  DelayLength=double(1)  InitialCondition=0  SampleTime=5e-07
  Delay_ValidIn : Delay  DelayLength=double(8)  InitialCondition=0  SampleTime=5e-07
  Discrete FIR Filter : Subsystem
  Enabled Wire : Subsystem
  FIR Scale : Gain  Gain="fi(0,1,19,20,\"hex\",\"20000\")"  ParamDataTypeStr=fixdt(1, 19, 20)  OutDataTypeStr=fixdt(1, 19, 18)  SampleTime=5e-07
  HDL Counter2 : Delay  DelayLength=double(1)  InitialCondition=0  SampleTime=5e-07
  Initial_ValAng : Constant  Value=0  OutDataTypeStr=fixdt(1, 19, 18)  SampleTime=5e-07
  Iteration : Subsystem
  Iteration1 : Subsystem
  Iteration2 : Subsystem
  Iteration3 : Subsystem
  Iteration4 : Subsystem
  Iteration_term0 : Terminator
  Iteration_term1 : Terminator
  Luise Scale : Gain  Gain="fi(0,1,19,10,\"hex\",\"40fc1\")"  ParamDataTypeStr=fixdt(1, 19, 10)  OutDataTypeStr=int16  SampleTime=5e-07
  Math Function1 : Math  Operator=conj  SignedPower=on  OutputSignalType=complex  OutDataTypeStr=fixdt(1, 16, 15)
  Output Register : Delay  DelayLength=double(1)  InitialCondition=0  SampleTime=5e-07
  Pipeline{1..5,11..12,21..22,31..32,41..42} (13 alike) : Delay  DelayLength=double(1)  InitialCondition=0  SampleTime=5e-07
  Product : Product  Inputs=**  OutDataTypeStr=fixdt(1, 32, 31)  SampleTime=5e-07
  QuadrantCorrection : Subsystem
  QuadrantMapper : Subsystem
  Raise to Power 4 : Subsystem
  SEL2 : MultiPortSwitch  DataPortOrder=Zero-based contiguous  Inputs=2  DiagnosticForDefault=None  zeroidx=on  OutDataTypeStr=fixdt(1, 32, 28)  SampleTime=5e-07  SaturateOnIntegerOverflow=off  InputSameDT=off
  Signal Specification : SignalSpecification  OutDataTypeStr=fixdt(1, 32, 31)  Dimensions=1
  Unit Delay1 : Delay  DelayLength=double(1)  InitialCondition=0  SampleTime=5e-07
  adder : Sum  OutDataTypeStr=fixdt(0, 12, 0)  AccumDataTypeStr=fixdt(0, 12, 0)  SampleTime=5e-07
  compare : simulink/Logic and Bit Operations/Compare To Constant  relop===  const="fi(0,0,12,0,\"hex\",\"0ff\")"  OutDataTypeStr=boolean
  const : Constant  Value=0.07798004150390625  OutDataTypeStr=fixdt(0, 16, 18)  SampleTime=5e-07
  const1 : Constant  Value=0.039585113525390625  OutDataTypeStr=fixdt(0, 16, 18)  SampleTime=5e-07
  const2 : Constant  Value=0.019866943359375  OutDataTypeStr=fixdt(0, 16, 18)  SampleTime=5e-07
  const3 : Constant  Value=0.009944915771484375  OutDataTypeStr=fixdt(0, 16, 18)  SampleTime=5e-07
  const4 : Constant  Value=0.1475830078125  OutDataTypeStr=fixdt(0, 16, 18)  SampleTime=5e-07
  const5 : Constant  Value=0  OutDataTypeStr=fixdt(1, 19, 18)  SampleTime=5e-07
  countFrom : Constant  Value=0  VectorParams1D=off  OutDataTypeStr=fixdt(0, 12, 0)  SampleTime=5e-07
  cplx2reim : ComplexToRealImag  SampleTime=5e-07
  dtc : DataTypeConversion  OutDataTypeStr=fixdt(1, 17, 13)  SampleTime=5e-07  SaturateOnIntegerOverflow=off  RndMeth=Floor
  dtc1 : DataTypeConversion  OutDataTypeStr=fixdt(1, 17, 13)  SampleTime=5e-07  SaturateOnIntegerOverflow=off  RndMeth=Floor
  invert_reset : simulink/Logic and Bit Operations/Bitwise Operator  logicop=NOT  UseBitMask=off  BitMask=double(0)  BitMaskRealWorld=Real World Value
  muxAng : Switch  Criteria=u2 ~= 0  Threshold="fi(0,0,1,0,\"hex\",\"0\")"  OutDataTypeStr=fixdt(1, 19, 18)  SampleTime=5e-07  SaturateOnIntegerOverflow=off  InputSameDT=off
  shift0 : Constant  VectorParams1D=off  OutDataTypeStr=fixdt(0, 4, 0)  SampleTime=5e-07
  shift1 : Constant  Value=2  VectorParams1D=off  OutDataTypeStr=fixdt(0, 4, 0)  SampleTime=5e-07
  shift2 : Constant  Value=3  VectorParams1D=off  OutDataTypeStr=fixdt(0, 4, 0)  SampleTime=5e-07
  shift3 : Constant  Value=4  VectorParams1D=off  OutDataTypeStr=fixdt(0, 4, 0)  SampleTime=5e-07
  shift4 : Constant  Value=5  VectorParams1D=off  OutDataTypeStr=fixdt(0, 4, 0)  SampleTime=5e-07
  step_value : Constant  VectorParams1D=off  OutDataTypeStr=fixdt(0, 12, 0)  SampleTime=5e-07
  switch : Switch  Criteria=u2 ~= 0  Threshold="fi(0,0,1,0,\"hex\",\"0\")"  OutDataTypeStr=fixdt(0, 12, 0)  SampleTime=5e-07  SaturateOnIntegerOverflow=off  InputSameDT=off
  zout_corrected_wire : hdlmdlgenlib/Buffer
  Estimate : Outport  SampleTime=5e-07  VectorParamsAs1DForOutWhenUnconnected=off
  Estimate Valid : Outport  Port=2  SampleTime=5e-07  VectorParamsAs1DForOutWhenUnconnected=off
  wires:
  QuadrantCorrection/1(zout) -> muxAng/3
  Compare To Constant2/1 -> Enabled Wire/2(Enable), Delay2/1, SEL2/1
  dataIn/1 -> Raise to Power 4/1(In1)
  Discrete FIR Filter/1(Discrete FIR Filter_out) -> FIR Scale/1
  Iteration/1(xout) -> Pipeline2/1
  DelayImagInput/1 -> QuadrantMapper/2(yin)
  countFrom/1 -> switch/1
  Iteration1/3(zout) -> Pipeline32/1
  Raise to Power 4/1(Out1) -> Math Function1/1, Delay5/1
  Delay5/1 -> Delay11/1
  Math Function1/1 -> Delay4/1
  QuadrantMapper/3(QA_Control) -> DelayQC_Control/1
  step_value/1 -> adder/2
  Iteration/2(yout) -> Pipeline21/1
  Delay4/1 -> Discrete FIR Filter/1(Discrete FIR Filter_in)
  Delay11/1 -> Product/2
  switch/1 -> HDL Counter2/1
  Delay12/1 -> Add2/2
  const1/1 -> Iteration1/4(lut_value)
  FIR Scale/1 -> Delay8/1
  HDL Counter2/1 -> adder/1, compare/1, Compare To Constant2/1
  Delay8/1 -> Product/1
  DelayQC_Control/1 -> QuadrantCorrection/2(QA_Control)
  compare/1 -> switch/2
  adder/1 -> switch/3
  Unit Delay1/1 -> Accum Scale/1, SEL2/2
  Constant1/1 -> SEL2/3
  Product/1 -> Delay12/1
  Delay3/1 -> Delay10/1
  Accum Scale/1 -> Enabled Wire/1(In1)
  Delay2/1 -> Delay3/1
  SEL2/1 -> Add2/1
  Enabled Wire/1(Out1) -> Signal Specification/1
  Add2/1 -> Unit Delay1/1
  Data Type Conversion/1 -> cplx2reim/1
  Signal Specification/1 -> Data Type Conversion/1
  Delay10/1 -> Estimate Valid/1
  shift2/1 -> Iteration1/5(idx)
  cplx2reim/2 -> dtc1/1
  cplx2reim/1 -> dtc/1
  dtc/1 -> DelayRealInput/1
  dtc1/1 -> DelayImagInput/1
  DelayRealInput/1 -> QuadrantMapper/1(xin)
  Output Register/1 -> zout_corrected_wire/1
  QuadrantMapper/1(xout) -> DelayQuadMapper1/1
  Pipeline32/1 -> Iteration2/3(zin)
  QuadrantMapper/2(yout) -> DelayQuadMapper2/1
  DelayQuadMapper2/1 -> Iteration4/2(yin)
  DelayQuadMapper1/1 -> Iteration4/1(xin)
  const5/1 -> Iteration4/3(zin)
  Iteration/3(zout) -> Pipeline22/1
  Pipeline1/1 -> Iteration/1(xin)
  shift0/1 -> Iteration4/5(idx)
  const4/1 -> Iteration4/4(lut_value)
  Iteration1/1(xout) -> Pipeline3/1
  Iteration4/1(xout) -> Pipeline1/1
  Pipeline2/1 -> Iteration1/1(xin)
  Iteration4/2(yout) -> Pipeline11/1
  Iteration4/3(zout) -> Pipeline12/1
  Pipeline11/1 -> Iteration/2(yin)
  shift1/1 -> Iteration/5(idx)
  Pipeline12/1 -> Iteration/3(zin)
  Pipeline21/1 -> Iteration1/2(yin)
  const/1 -> Iteration/4(lut_value)
  Pipeline22/1 -> Iteration1/3(zin)
  Iteration1/2(yout) -> Pipeline31/1
  Pipeline3/1 -> Iteration2/1(xin)
  Pipeline31/1 -> Iteration2/2(yin)
  const2/1 -> Iteration2/4(lut_value)
  shift3/1 -> Iteration2/5(idx)
  Iteration2/1(xout) -> Pipeline4/1
  Initial_ValAng/1 -> muxAng/1
  Iteration2/2(yout) -> Pipeline41/1
  Iteration2/3(zout) -> Pipeline42/1
  Pipeline4/1 -> Iteration3/1(xin)
  Pipeline41/1 -> Iteration3/2(yin)
  Pipeline42/1 -> Iteration3/3(zin)
  const3/1 -> Iteration3/4(lut_value)
  shift4/1 -> Iteration3/5(idx)
  Constant/1 -> Delay_ValidIn/1
  Iteration3/1(xout) -> Iteration_term0/1
  Iteration3/2(yout) -> Iteration_term1/1
  Iteration3/3(zout) -> Pipeline5/1
  Delay_ValidIn/1 -> invert_reset/1
  Pipeline5/1 -> QuadrantCorrection/1(zin)
  invert_reset/1 -> muxAng/2
  muxAng/1 -> Output Register/1
  zout_corrected_wire/1 -> Delay1/1
  Delay1/1 -> Luise Scale/1
  Luise Scale/1 -> Delay9/1
  Delay9/1 -> Estimate/1
